simulink model "s_b4a4x2kf"  (R2016b)
settings: Solver=VariableStepDiscrete  StartTime=0.0  StopTime=1  RelTol=1e-3
undefined symbols (not defined in the file): fft_stages, n_bits_ants, n_bits_xengs
libraries: xbsIndex_r4 x16372, casper_library_misc x151, xbsReplacements_r4 x9, casper_library_delays x8, xps_library x3
(part 11 of 139)

== system s_b4a4x2kf/snap_pack_mux ==
  in_input_select : Inport
  in_eof : Inport  Port=2
  in_go0 : Inport  Port=3
  in_go1 : Inport  Port=4
  in_go2 : Inport  Port=5
  in_go3 : Inport  Port=6
  in_bf0_tx_pkt0 : Inport  Port=7
  in_bf0_tx_pkt1 : Inport  Port=8
  in_bf0_tx_pkt2 : Inport  Port=9
  in_bf0_tx_pkt3 : Inport  Port=10
  in_bf1_tx_pkt0 : Inport  Port=11
  in_bf1_tx_pkt1 : Inport  Port=12
  in_bf1_tx_pkt2 : Inport  Port=13
  in_bf1_tx_pkt3 : Inport  Port=14
  in_rdy0 : Inport  Port=15
  in_rdy1 : Inport  Port=16
  in_rdy2 : Inport  Port=17
  in_rdy3 : Inport  Port=18
  in_bf0_rdy0 : Inport  Port=19
  in_bf0_rdy1 : Inport  Port=20
  in_bf0_rdy2 : Inport  Port=21
  in_bf0_rdy3 : Inport  Port=22
  in_bf1_rdy0 : Inport  Port=23
  in_bf1_rdy1 : Inport  Port=24
  in_bf1_rdy2 : Inport  Port=25
  in_bf1_rdy3 : Inport  Port=26
  in_vld0 : Inport  Port=27
  in_vld1 : Inport  Port=28
  in_vld2 : Inport  Port=29
  in_vld3 : Inport  Port=30
  in_bf0_vld0 : Inport  Port=31
  in_bf0_vld1 : Inport  Port=32
  in_bf0_vld2 : Inport  Port=33
  in_bf0_vld3 : Inport  Port=34
  in_bf1_vld0 : Inport  Port=35
  in_bf1_vld1 : Inport  Port=36
  in_bf1_vld2 : Inport  Port=37
  in_bf1_vld3 : Inport  Port=38
  in_eof0 : Inport  Port=39
  in_eof1 : Inport  Port=40
  in_eof2 : Inport  Port=41
  in_eof3 : Inport  Port=42
  in_bf0_eof0 : Inport  Port=43
  in_bf0_eof1 : Inport  Port=44
  in_bf0_eof2 : Inport  Port=45
  in_bf0_eof3 : Inport  Port=46
  in_bf1_eof0 : Inport  Port=47
  in_bf1_eof1 : Inport  Port=48
  in_bf1_eof2 : Inport  Port=49
  in_bf1_eof3 : Inport  Port=50
  in_ip : Inport  Port=51
  we : Inport  Port=52
  trig : Inport  Port=53
  assert_bf0_eof{0..3} (4 alike) : xbsIndex_r4/Assert  assert_type=on  type_source=Explicitly  gui_display_data_type=Boolean  arith_type=Boolean  n_bits=1  bin_pt=0  preci_type=Single  exp_width=8  frac_width=24  assert_rate=off  rate_source=Explicitly  period=1  output_port=on  block_type=assert
  assert_bf0_rdy{0..3} (4 alike) : xbsIndex_r4/Assert  assert_type=on  type_source=Explicitly  gui_display_data_type=Boolean  arith_type=Boolean  n_bits=1  bin_pt=0  preci_type=Single  exp_width=8  frac_width=24  assert_rate=off  rate_source=Explicitly  period=1  output_port=on  block_type=assert
  assert_bf0_tx_pkt{0..3} (4 alike) : xbsIndex_r4/Assert  assert_type=on  type_source=Explicitly  gui_display_data_type=Boolean  arith_type=Boolean  n_bits=1  bin_pt=0  preci_type=Single  exp_width=8  frac_width=24  assert_rate=off  rate_source=Explicitly  period=1  output_port=on  block_type=assert
  assert_bf0_vld{0..3} (4 alike) : xbsIndex_r4/Assert  assert_type=on  type_source=Explicitly  gui_display_data_type=Boolean  arith_type=Boolean  n_bits=1  bin_pt=0  preci_type=Single  exp_width=8  frac_width=24  assert_rate=off  rate_source=Explicitly  period=1  output_port=on  block_type=assert
  assert_bf1_eof{0..3} (4 alike) : xbsIndex_r4/Assert  assert_type=on  type_source=Explicitly  gui_display_data_type=Boolean  arith_type=Boolean  n_bits=1  bin_pt=0  preci_type=Single  exp_width=8  frac_width=24  assert_rate=off  rate_source=Explicitly  period=1  output_port=on  block_type=assert
  assert_bf1_rdy{0..3} (4 alike) : xbsIndex_r4/Assert  assert_type=on  type_source=Explicitly  gui_display_data_type=Boolean  arith_type=Boolean  n_bits=1  bin_pt=0  preci_type=Single  exp_width=8  frac_width=24  assert_rate=off  rate_source=Explicitly  period=1  output_port=on  block_type=assert
  assert_bf1_tx_pkt{0..3} (4 alike) : xbsIndex_r4/Assert  assert_type=on  type_source=Explicitly  gui_display_data_type=Boolean  arith_type=Boolean  n_bits=1  bin_pt=0  preci_type=Single  exp_width=8  frac_width=24  assert_rate=off  rate_source=Explicitly  period=1  output_port=on  block_type=assert
  assert_bf1_vld{0..3} (4 alike) : xbsIndex_r4/Assert  assert_type=on  type_source=Explicitly  gui_display_data_type=Boolean  arith_type=Boolean  n_bits=1  bin_pt=0  preci_type=Single  exp_width=8  frac_width=24  assert_rate=off  rate_source=Explicitly  period=1  output_port=on  block_type=assert
  assert_eof{,0..3} (5 alike) : xbsIndex_r4/Assert  assert_type=on  type_source=Explicitly  gui_display_data_type=Boolean  arith_type=Boolean  n_bits=1  bin_pt=0  preci_type=Single  exp_width=8  frac_width=24  assert_rate=off  rate_source=Explicitly  period=1  output_port=on  block_type=assert
  assert_go{0..3} (4 alike) : xbsIndex_r4/Assert  assert_type=on  type_source=Explicitly  gui_display_data_type=Boolean  arith_type=Boolean  n_bits=1  bin_pt=0  preci_type=Single  exp_width=8  frac_width=24  assert_rate=off  rate_source=Explicitly  period=1  output_port=on  block_type=assert
  assert_input_select : xbsIndex_r4/Assert  assert_type=on  type_source=Explicitly  gui_display_data_type=Fixed-point  arith_type=Unsigned  n_bits=4  bin_pt=0  preci_type=Single  exp_width=8  frac_width=24  assert_rate=off  rate_source=Explicitly  period=1  output_port=on  block_type=assert
  assert_ip : xbsIndex_r4/Assert  assert_type=on  type_source=Explicitly  gui_display_data_type=Fixed-point  arith_type=Unsigned  n_bits=11  bin_pt=0  preci_type=Single  exp_width=8  frac_width=24  assert_rate=off  rate_source=Explicitly  period=1  output_port=on  block_type=assert
  assert_rdy{0..3} (4 alike) : xbsIndex_r4/Assert  assert_type=on  type_source=Explicitly  gui_display_data_type=Boolean  arith_type=Boolean  n_bits=1  bin_pt=0  preci_type=Single  exp_width=8  frac_width=24  assert_rate=off  rate_source=Explicitly  period=1  output_port=on  block_type=assert
  assert_vld{0..3} (4 alike) : xbsIndex_r4/Assert  assert_type=on  type_source=Explicitly  gui_display_data_type=Boolean  arith_type=Boolean  n_bits=1  bin_pt=0  preci_type=Single  exp_width=8  frac_width=24  assert_rate=off  rate_source=Explicitly  period=1  output_port=on  block_type=assert
  buscreate : Subsystem  AncestorBlock=casper_library_flow_control/bus_create  mask(bus_create){inputNum=51}
      mask prompts: inputNum "Number of inputs:"
      mask init:
      | bus_create_init(gcb,...
      |     'inputNum', inputNum);
  io_delay : Subsystem  AncestorBlock=casper_library_delays/pipeline  mask(pipeline){latency=2}
      mask help:
      | An explicitly laid-out delay line to avoid mapping to SRL16s
      | for use in pipelining to help achieve timing closure.
      mask init:
      | pipeline_init(gcb,'latency',latency);
      settings: AttributesFormatString=Latency = %<latency>
      mask Display:
      | port_label('input', 1, 'd');
      | port_label('output', 1, 'q');
      | disp(['Z^-', num2str(latency)]);
  ss : Subsystem  Tag=casper:snapshot  AncestorBlock=casper_library_scopes/snapshot  mask(snapshot){storage=bram, dram_dimm=2, dram_clock=250, nsamples=12, data_width=64, offset=off, circap=off, value=off, ext_arm=off, ext_circ=off, provide_outputs=off, use_dsp48=on}
      mask prompts: storage "Storage medium"; dram_dimm "DRAM dimm"; dram_clock "DRAM clock rate"; nsamples "Number of Samples (2^?)"; data_width "Data width"; offset "Start delay support"; circap "Circular capture support"; value "Extra value capture support"; ext_arm "External arm support"; ext_circ "External circular capture support"; provide_outputs "Provide outputs"; use_dsp48 "Use DSP48s to implement counters"
      mask help:
      | Standard snap block, but with the following optional extras;
      |  1) Optionally delay the fabric trigger by a user-specified number of valids.
      |  2) Capture continuously after a trigger until a stop pulse is received. Data is captured into BRAM continuously, with old data being overwritten until a stop command is received. Then stop capturing when memory is filled. This enables you to get some data before and some data after the stop pulse. Use the 'tr_en_cnt' register to determine where you are in your vector. 'Addr' register's MSb now indicates 'busy capturing'.
      |  3) Optionally capture a value on an input port to a register at the same time as the first data sample.
      |  4) Implement counters using DSP48Es to save resources.
      mask init:
      | snapshot_init(gcb, ...
      |     'storage', storage, ...
      |     'dram_dimm', dram_dimm, ...
      |     'dram_clock', dram_clock, ...
      |     'nsamples', nsamples, ...
      |     'data_width', data_width, ...
      |     'offset', offset, ...
      |     'circap', circap, ...
      |     'value', value, ...
      |     'ext_arm', ext_arm, ...
      |     'ext_circ', ext_circ, ...
      |     'provide_outputs', 'off', ...
      |     'use_dsp48', use_dsp48);
      settings: AttributesFormatString=|
      | 64 wide, 4096 deep
      | debugID: 28962935
      mask TypeOptions storage: bram | dram
      mask Callback storage: snapshot_callback();
      mask TypeOptions dram_dimm: 1 | 2 | 3 | 4
      mask TypeOptions dram_clock: 200 | 250 | 266 | 300 | 333
      mask TypeOptions data_width: 8 | 16 | 32 | 64 | 128
  trig_delay : Subsystem  AncestorBlock=casper_library_delays/pipeline  mask(pipeline){latency=2}
      mask help:
      | An explicitly laid-out delay line to avoid mapping to SRL16s
      | for use in pipelining to help achieve timing closure.
      mask init:
      | pipeline_init(gcb,'latency',latency);
      settings: AttributesFormatString=Latency = %<latency>
      mask Display:
      | port_label('input', 1, 'd');
      | port_label('output', 1, 'q');
      | disp(['Z^-', num2str(latency)]);
  we_delay : Subsystem  AncestorBlock=casper_library_delays/pipeline  mask(pipeline){latency=2}
      mask help:
      | An explicitly laid-out delay line to avoid mapping to SRL16s
      | for use in pipelining to help achieve timing closure.
      mask init:
      | pipeline_init(gcb,'latency',latency);
      settings: AttributesFormatString=Latency = %<latency>
      mask Display:
      | port_label('input', 1, 'd');
      | port_label('output', 1, 'q');
      | disp(['Z^-', num2str(latency)]);
  arm_out : Outport
  wires:
  ss/1(arm_out) -> arm_out/1
  buscreate/1(bus_out) -> io_delay/1(d)
  io_delay/1(q) -> ss/1(din)
  in_input_select/1 -> assert_input_select/1
  assert_input_select/1 -> buscreate/1(in1)
  in_eof/1 -> assert_eof/1
  assert_eof/1 -> buscreate/2(in2)
  in_go0/1 -> assert_go0/1
  assert_go0/1 -> buscreate/3(in3)
  in_go1/1 -> assert_go1/1
  assert_go1/1 -> buscreate/4(in4)
  in_go2/1 -> assert_go2/1
  assert_go2/1 -> buscreate/5(in5)
  in_go3/1 -> assert_go3/1
  assert_go3/1 -> buscreate/6(in6)
  in_bf0_tx_pkt0/1 -> assert_bf0_tx_pkt0/1
  assert_bf0_tx_pkt0/1 -> buscreate/7(in7)
  in_bf0_tx_pkt1/1 -> assert_bf0_tx_pkt1/1
  assert_bf0_tx_pkt1/1 -> buscreate/8(in8)
  in_bf0_tx_pkt2/1 -> assert_bf0_tx_pkt2/1
  assert_bf0_tx_pkt2/1 -> buscreate/9(in9)
  in_bf0_tx_pkt3/1 -> assert_bf0_tx_pkt3/1
  assert_bf0_tx_pkt3/1 -> buscreate/10(in10)
  in_bf1_tx_pkt0/1 -> assert_bf1_tx_pkt0/1
  assert_bf1_tx_pkt0/1 -> buscreate/11(in11)
  in_bf1_tx_pkt1/1 -> assert_bf1_tx_pkt1/1
  assert_bf1_tx_pkt1/1 -> buscreate/12(in12)
  in_bf1_tx_pkt2/1 -> assert_bf1_tx_pkt2/1
  assert_bf1_tx_pkt2/1 -> buscreate/13(in13)
  in_bf1_tx_pkt3/1 -> assert_bf1_tx_pkt3/1
  assert_bf1_tx_pkt3/1 -> buscreate/14(in14)
  in_rdy0/1 -> assert_rdy0/1
  assert_rdy0/1 -> buscreate/15(in15)
  in_rdy1/1 -> assert_rdy1/1
  assert_rdy1/1 -> buscreate/16(in16)
  in_rdy2/1 -> assert_rdy2/1
  assert_rdy2/1 -> buscreate/17(in17)
  in_rdy3/1 -> assert_rdy3/1
  assert_rdy3/1 -> buscreate/18(in18)
  in_bf0_rdy0/1 -> assert_bf0_rdy0/1
  assert_bf0_rdy0/1 -> buscreate/19(in19)
  in_bf0_rdy1/1 -> assert_bf0_rdy1/1
  assert_bf0_rdy1/1 -> buscreate/20(in20)
  in_bf0_rdy2/1 -> assert_bf0_rdy2/1
  assert_bf0_rdy2/1 -> buscreate/21(in21)
  in_bf0_rdy3/1 -> assert_bf0_rdy3/1
  assert_bf0_rdy3/1 -> buscreate/22(in22)
  in_bf1_rdy0/1 -> assert_bf1_rdy0/1
  assert_bf1_rdy0/1 -> buscreate/23(in23)
  in_bf1_rdy1/1 -> assert_bf1_rdy1/1
  assert_bf1_rdy1/1 -> buscreate/24(in24)
  in_bf1_rdy2/1 -> assert_bf1_rdy2/1
  assert_bf1_rdy2/1 -> buscreate/25(in25)
  in_bf1_rdy3/1 -> assert_bf1_rdy3/1
  assert_bf1_rdy3/1 -> buscreate/26(in26)
  in_vld0/1 -> assert_vld0/1
  assert_vld0/1 -> buscreate/27(in27)
  in_vld1/1 -> assert_vld1/1
  assert_vld1/1 -> buscreate/28(in28)
  in_vld2/1 -> assert_vld2/1
  assert_vld2/1 -> buscreate/29(in29)
  in_vld3/1 -> assert_vld3/1
  assert_vld3/1 -> buscreate/30(in30)
  in_bf0_vld0/1 -> assert_bf0_vld0/1
  assert_bf0_vld0/1 -> buscreate/31(in31)
  in_bf0_vld1/1 -> assert_bf0_vld1/1
  assert_bf0_vld1/1 -> buscreate/32(in32)
  in_bf0_vld2/1 -> assert_bf0_vld2/1
  assert_bf0_vld2/1 -> buscreate/33(in33)
  in_bf0_vld3/1 -> assert_bf0_vld3/1
  assert_bf0_vld3/1 -> buscreate/34(in34)
  in_bf1_vld0/1 -> assert_bf1_vld0/1
  assert_bf1_vld0/1 -> buscreate/35(in35)
  in_bf1_vld1/1 -> assert_bf1_vld1/1
  assert_bf1_vld1/1 -> buscreate/36(in36)
  in_bf1_vld2/1 -> assert_bf1_vld2/1
  assert_bf1_vld2/1 -> buscreate/37(in37)
  in_bf1_vld3/1 -> assert_bf1_vld3/1
  assert_bf1_vld3/1 -> buscreate/38(in38)
  in_eof0/1 -> assert_eof0/1
  assert_eof0/1 -> buscreate/39(in39)
  in_eof1/1 -> assert_eof1/1
  assert_eof1/1 -> buscreate/40(in40)
  in_eof2/1 -> assert_eof2/1
  assert_eof2/1 -> buscreate/41(in41)
  in_eof3/1 -> assert_eof3/1
  assert_eof3/1 -> buscreate/42(in42)
  in_bf0_eof0/1 -> assert_bf0_eof0/1
  assert_bf0_eof0/1 -> buscreate/43(in43)
  in_bf0_eof1/1 -> assert_bf0_eof1/1
  assert_bf0_eof1/1 -> buscreate/44(in44)
  in_bf0_eof2/1 -> assert_bf0_eof2/1
  assert_bf0_eof2/1 -> buscreate/45(in45)
  in_bf0_eof3/1 -> assert_bf0_eof3/1
  assert_bf0_eof3/1 -> buscreate/46(in46)
  in_bf1_eof0/1 -> assert_bf1_eof0/1
  assert_bf1_eof0/1 -> buscreate/47(in47)
  in_bf1_eof1/1 -> assert_bf1_eof1/1
  assert_bf1_eof1/1 -> buscreate/48(in48)
  in_bf1_eof2/1 -> assert_bf1_eof2/1
  assert_bf1_eof2/1 -> buscreate/49(in49)
  in_bf1_eof3/1 -> assert_bf1_eof3/1
  assert_bf1_eof3/1 -> buscreate/50(in50)
  in_ip/1 -> assert_ip/1
  assert_ip/1 -> buscreate/51(in51)
  we/1 -> we_delay/1(d)
  we_delay/1(q) -> ss/2(we)
  trig/1 -> trig_delay/1(d)
  trig_delay/1(q) -> ss/3(trig)

== system s_b4a4x2kf/spead_status ==
  out_magic_err_cnt : Inport
  out_header_err_cnt : Inport  Port=2
  out_pad_err_cnt : Inport  Port=3
  out_pkt_len_err_cnt : Inport  Port=4
  out_pkt_cnt : Inport  Port=5
  assert_header_err_cnt : xbsIndex_r4/Assert  assert_type=on  type_source=Explicitly  gui_display_data_type=Fixed-point  arith_type=Unsigned  n_bits=6  bin_pt=0  preci_type=Single  exp_width=8  frac_width=24  assert_rate=off  rate_source=Explicitly  period=1  output_port=on  block_type=assert
  assert_magic_err_cnt : xbsIndex_r4/Assert  assert_type=on  type_source=Explicitly  gui_display_data_type=Fixed-point  arith_type=Unsigned  n_bits=6  bin_pt=0  preci_type=Single  exp_width=8  frac_width=24  assert_rate=off  rate_source=Explicitly  period=1  output_port=on  block_type=assert
  assert_pad_err_cnt : xbsIndex_r4/Assert  assert_type=on  type_source=Explicitly  gui_display_data_type=Fixed-point  arith_type=Unsigned  n_bits=6  bin_pt=0  preci_type=Single  exp_width=8  frac_width=24  assert_rate=off  rate_source=Explicitly  period=1  output_port=on  block_type=assert
  assert_pkt_cnt : xbsIndex_r4/Assert  assert_type=on  type_source=Explicitly  gui_display_data_type=Fixed-point  arith_type=Unsigned  n_bits=6  bin_pt=0  preci_type=Single  exp_width=8  frac_width=24  assert_rate=off  rate_source=Explicitly  period=1  output_port=on  block_type=assert
  assert_pkt_len_err_cnt : xbsIndex_r4/Assert  assert_type=on  type_source=Explicitly  gui_display_data_type=Fixed-point  arith_type=Unsigned  n_bits=6  bin_pt=0  preci_type=Single  exp_width=8  frac_width=24  assert_rate=off  rate_source=Explicitly  period=1  output_port=on  block_type=assert
  cast_gw : xbsIndex_r4/Convert  gui_display_data_type=Fixed-point  arith_type=Unsigned  n_bits=32  bin_pt=0  float_type=Single  exp_bits=8  fraction_bits=24  quantization=Truncate  overflow=Wrap  en=off  latency=1  pipeline=off  dbl_ovrd=off  block_type=convert
  concatenate : xbsIndex_r4/Concat  num_inputs=5  dbl_ovrd=off  block_type=concat
  io_delay : xbsIndex_r4/Delay  rst=off  infoeditControl=Selection of Reset will increase slice count due to use of real FFs and instead of SRLs  en=off  latency=0  reg_retiming=on  dbl_ovrd=off  block_type=delay
      settings: infoedit=Hardware notes: A delay line is a chain, each link of which is an SRL16 or SRL32 followed by a flip-flop.
  reint{1..5} (5 alike) : xbsIndex_r4/Reinterpret  force_arith_type=on  arith_type=Unsigned  force_bin_pt=on  bin_pt=0  block_type=reinterpret
  s_b4a4x2kf_spead_status_user_data_in : xbsIndex_r4/Gateway Out  inherit_from_input=off  hdl_port=on  rows=1  columns=1  UseAsDAC=off  DACChannel='1'  interface=None  automatic_assignment=on  address_offset=hex2dec('00')  intf_name=''  intf_description=''  timing_constraint=None  locs_specified=off  LOCs={}  io_standard={}  block_type=gatewayout
  sim_out : Terminator
  wires:
  concatenate/1 -> io_delay/1
  io_delay/1 -> cast_gw/1
  cast_gw/1 -> s_b4a4x2kf_spead_status_user_data_in/1
  s_b4a4x2kf_spead_status_user_data_in/1 -> sim_out/1
  out_magic_err_cnt/1 -> assert_magic_err_cnt/1
  assert_magic_err_cnt/1 -> reint1/1
  reint1/1 -> concatenate/1
  out_header_err_cnt/1 -> assert_header_err_cnt/1
  assert_header_err_cnt/1 -> reint2/1
  reint2/1 -> concatenate/2
  out_pad_err_cnt/1 -> assert_pad_err_cnt/1
  assert_pad_err_cnt/1 -> reint3/1
  reint3/1 -> concatenate/3
  out_pkt_len_err_cnt/1 -> assert_pkt_len_err_cnt/1
  assert_pkt_len_err_cnt/1 -> reint4/1
  reint4/1 -> concatenate/4
  out_pkt_cnt/1 -> assert_pkt_cnt/1
  assert_pkt_cnt/1 -> reint5/1
  reint5/1 -> concatenate/5

== system s_b4a4x2kf/spead_time_check ==
  Constant : xbsIndex_r4/Constant  const=0  gui_display_data_type=Fixed-point  arith_type=Unsigned  n_bits=12  bin_pt=0  preci_type=Single  exp_width=8  frac_width=24  explicit_period=on  period=1  equ=P=C  opselect=C  inp2=PCIN>>17  opr=+  inp1=P  carry=CIN  dbl_ovrd=off  block_type=constant
  Counter : xbsIndex_r4/Counter  cnt_type=Free Running  cnt_to=Inf  operation=Up  start_count=0  cnt_by_val=1  arith_type=Unsigned  n_bits=16  bin_pt=0  load_pin=off  rst=on  en=on  explicit_period=on  period=1  use_behavioral_HDL=on  implementation=Fabric  dbl_ovrd=off  block_type=counter
  Delay : xbsIndex_r4/Delay  rst=off  infoeditControl=Selection of Reset will increase slice count due to use of real FFs and instead of SRLs  en=off  latency=1  reg_retiming=on  dbl_ovrd=off  block_type=delay
  Delay41 : Subsystem  AncestorBlock=casper_library_delays/pipeline  mask(pipeline){latency=2}
      mask help:
      | An explicitly laid-out delay line to avoid mapping to SRL16s
      | for use in pipelining to help achieve timing closure.
      mask init:
      | pipeline_init(gcb,'latency',latency);
      settings: AttributesFormatString=Latency = %<latency>
      mask Display:
      | port_label('input', 1, 'd');
      | port_label('output', 1, 'q');
      | disp(['Z^-', num2str(latency)]);
  Delay8 : Subsystem  AncestorBlock=casper_library_delays/pipeline  mask(pipeline){latency=2}
      mask help:
      | An explicitly laid-out delay line to avoid mapping to SRL16s
      | for use in pipelining to help achieve timing closure.
      mask init:
      | pipeline_init(gcb,'latency',latency);
      settings: AttributesFormatString=Latency = %<latency>
      mask Display:
      | port_label('input', 1, 'd');
      | port_label('output', 1, 'q');
      | disp(['Z^-', num2str(latency)]);
  Logical6 : xbsIndex_r4/Logical  logical_function=AND  inputs=2  en=off  latency=0  precision=Full  arith_type=Unsigned  n_bits=16  bin_pt=0  align_bp=on  dbl_ovrd=off  block_type=logical
  Relational : xbsIndex_r4/Relational  mode=a!=b  op_type=Bool  en=off  latency=1  dbl_ovrd=off  block_type=relational
  Slice5 : xbsIndex_r4/Slice  nbits=12  boolean_output=off  mode=Lower Bit Location + Width  bit1=0  base1=MSB of Input  bit0=0  base0=LSB of Input  dbl_ovrd=off  block_type=slice
  lsbzero0 : Outport
  wires:
  Delay8/1(q) -> lsbzero0/1
  Slice5/1 -> Relational/2
  Constant/1 -> Relational/1
  Relational/1 -> Logical6/2
  Delay/1 -> Logical6/1
  Logical6/1 -> Counter/2
  [cnt_rst] -> Delay41/1(d)
  Delay41/1(q) -> Counter/1
  Counter/1 -> Delay8/1(d)
  [spead_valid] -> Delay/1
  [spead_timestamp] -> Slice5/1

== system s_b4a4x2kf/speadtime_lsbzero ==
  out_spead0 : Inport
  assert_spead0 : xbsIndex_r4/Assert  assert_type=on  type_source=Explicitly  gui_display_data_type=Fixed-point  arith_type=Unsigned  n_bits=16  bin_pt=0  preci_type=Single  exp_width=8  frac_width=24  assert_rate=off  rate_source=Explicitly  period=1  output_port=on  block_type=assert
  cast_gw : xbsIndex_r4/Convert  gui_display_data_type=Fixed-point  arith_type=Unsigned  n_bits=32  bin_pt=0  float_type=Single  exp_bits=8  fraction_bits=24  quantization=Truncate  overflow=Wrap  en=off  latency=1  pipeline=off  dbl_ovrd=off  block_type=convert
  io_delay : xbsIndex_r4/Delay  rst=off  infoeditControl=Selection of Reset will increase slice count due to use of real FFs and instead of SRLs  en=off  latency=0  reg_retiming=on  dbl_ovrd=off  block_type=delay
      settings: infoedit=Hardware notes: A delay line is a chain, each link of which is an SRL16 or SRL32 followed by a flip-flop.
  reint1 : xbsIndex_r4/Reinterpret  force_arith_type=on  arith_type=Unsigned  force_bin_pt=on  bin_pt=0  block_type=reinterpret
  s_b4a4x2kf_speadtime_lsbzero_user_data_in : xbsIndex_r4/Gateway Out  inherit_from_input=off  hdl_port=on  rows=1  columns=1  UseAsDAC=off  DACChannel='1'  interface=None  automatic_assignment=on  address_offset=hex2dec('00')  intf_name=''  intf_description=''  timing_constraint=None  locs_specified=off  LOCs={}  io_standard={}  block_type=gatewayout
  sim_out : Terminator
  wires:
  io_delay/1 -> cast_gw/1
  cast_gw/1 -> s_b4a4x2kf_speadtime_lsbzero_user_data_in/1
  s_b4a4x2kf_speadtime_lsbzero_user_data_in/1 -> sim_out/1
  out_spead0/1 -> assert_spead0/1
  assert_spead0/1 -> reint1/1
  reint1/1 -> io_delay/1
